simulink model "sm_car_"  (R2026b)
settings: Solver=ode23t  StopTime=100  MaxStep=0.4  AbsTol=1e-3  EnableMultiTasking=on
PreLoadFcn:
  | % Due to usability issue in Repeating Sequence block
  | warning('off','Simulink:Masking:Invalid');
  | 
  | % Eliminate unnecessary warnings in inactive variants
  | % Warnings generated only if you click through inactive variant
  | warning('off','MATLAB:nonExistentField');
  | warning('off','Simulink:Parameters:BlkParamUndefined');
PostLoadFcn:
  | set_param([bdroot '/Vehicle'],'popup_trailer','Off')
  | warning('off','sm:sli:setup:compile:LocalSolverNotSupported')
  | %sm_car_config_maneuver(bdroot,'WOT Braking');
  | sm_car_config_vehicle(bdroot,'false');
  | sm_car_config_logging(bdroot);
InitFcn:
  | sm_car_config_camera;
  | Vehicle = sm_car_vehcfg_checkConfig(Vehicle);
  | sm_car_check_tire_model(bdroot);
StartFcn:
  | tic;
StopFcn:
  | Elapsed_Sim_Time = toc;
  | % disp(['Elapsed Sim Time = ' num2str(Elapsed_Sim_Time)]);
undefined symbols (not defined in the file or in its folder): acc_theta, accel_ramp_rate, Axle1D, AxleIn, Camera, Control, Driver, Init, Maneuver, Pedal, Scene, ShaftL1, ShaftL2, ShaftR1, ShaftR2, Visual, X, xy_data_car_side, Y, Z
libraries: sm_lib x290, fl_lib x171, nesl_utility x144, simulink x60, simulink_extras x14, sdl_lib x14, SimscapeFluids_lib x7, Damper_Element x4, Tire_1x2x x4, ee_lib x3, Scene_Utilities x3, sharedTrackingLibrary x2
(part 4 of 22)

== system sm_car_/Controller/TrqVec_FLC_V3 ==
  DrvBus : Inport
  VehBus : Inport  Port=2
  Brake Control : Subsystem  Variant=on  VariantControlMode=label  VariantControl=Variant1  LabelModeActiveChoice=Pedal  mask{popup_brake_control=Pedal, abs_tire_radiusF=Vehicle.Chassis.Tire.tire_radius.Value, abs_tire_radiusR=Vehicle.Chassis.Tire.tire_radius.Value}
      mask prompts: popup_brake_control "Control Type"; abs_tire_radiusF "Tire Radius Front (m)"; abs_tire_radiusR "Tire Radius Rear (m)"
      mask init:
      | set_param(gcb,'LabelModeActiveChoice',get_param(gcb,'popup_brake_control'));
      settings: AttributesFormatString=%<ActiveVariant>
      mask TypeOptions popup_brake_control: Pedal | Pressure | ABS
      mask Display: disp(' ');
  Bus Creator1 : BusCreator  Inputs=4
  Bus Creator2 : BusCreator  Inputs=6
  Bus Selector : BusSelector  OutputSignals=Chassis.Body.CG.vx
  Bus Selector1 : BusSelector  OutputSignals=aSteerWheel,rAccelPedal,rBrakePedal
  Driveline Control : Subsystem
  Power Control : Subsystem  mask{Control=Control}
      mask prompts: Control "Control Parameters"
  Spring Damper : Subsystem
  Susp : Subsystem  mask{Steer=Control.Steer}
      mask prompts: Steer "Steer (structure)"
  CtrlBus : Outport  VectorParamsAs1DForOutWhenUnconnected=off
  wires:
  DrvBus/1 -> Bus Selector1/1
  Bus Creator2/1 -> CtrlBus/1  "CtrlBus"
  Bus Selector1/3 -> Brake Control/1("rBrakePedal ")  "<rBrakePedal>"
  Bus Selector1/2 -> Power Control/1(rAccelPedal)  "<rAccelPedal>"
  Spring Damper/2(Spring) -> Bus Creator1/4
  Power Control/1(Power) -> Bus Creator2/2  "Power"
  Driveline Control/1(Driveline) -> Bus Creator2/4
  Spring Damper/1(Damper) -> Bus Creator1/3
  Bus Creator1/1 -> Bus Creator2/1  "Chassis"
  Brake Control/1(" Brakes") -> Bus Creator2/5
  Susp/1(SuspA1) -> Bus Creator1/1
  VehBus/1 -> Power Control/2(VehBus), Brake Control/2("VehBus "), Bus Selector/1
  Susp/2(SuspA2) -> Bus Creator1/2
  Bus Selector1/1 -> Power Control/3(aSteerWheel), Susp/1(aSteerWheel)  "<aSteerWheel>"
  Bus Selector/1 -> Susp/2(vx)  "<vx>"
  Power Control/2(Meas) -> Bus Creator2/3  "Control"

== system sm_car_/Driver/Closed Loop ==
  VehBus : Inport
  Obs : Inport  Port=2
  Bus Selector : BusSelector  OutputSignals=Chassis.Body.CG.vx
  Bus Selector2 : BusSelector  OutputSignals=dist
  Driver : Subsystem  mask(Driver Behavior){Driver=Driver}
      mask help: Models driver behavior to follow prescribed vehicle trajectory, including path and speed.
  Driver Override : Subsystem  Variant=on  VariantControlMode=label  VariantControl=Choice  LabelModeActiveChoice=None  mask(Override Driver Commands){popup_driver_override=None}
      mask prompts: popup_driver_override "Driver Override"
      mask help: Override closed-loop driver commands with open-loop inputs. Can be applied to steering wheel, accelerator pedal. or brake pedal.
      mask init:
      | curblk = gcb;
      | 
      | set_param(curblk,'LabelModeActiveChoice',get_param(curblk,'popup_driver_override'));
      mask TypeOptions popup_driver_override: None | Override
  Maneuver : Subsystem  mask(Maneuver Follow Trajectory){Maneuver=Maneuver, Value=Maneuver.vGain.Value, popup_window=Yes}
      mask prompts: Value "vGain"; popup_window "Check only window of trajectory"
      mask help: Determines target pose to follow prescribed trajectory. Prescribed trajectory is vehicle pose (x, y, theta) and speed along the path to be followed. Optional visual of target pose is also provided.
      mask init:
      | if(strcmpi(get_param(gcb,'popup_window'),'yes'))
      |     set_param([gcb '/window only'],'Value','1');
      | else
      |     set_param([gcb '/window only'],'Value','0');
      | end
      mask TypeOptions Value: Target Speed Gain/Value
      mask TypeOptions popup_window: No | Yes
  Override : Subsystem  Variant=on  VariantControlMode=label  VariantControl=Variant1  LabelModeActiveChoice=None  mask(Driver Override){popup_override_type=None}
      mask prompts: popup_override_type "Override Type"
      mask help: Optionally override driver commands based on objects in scene. For example, the state of a traffic light can override driver commands to follow a prescribed speed trajectory.
      mask init:
      | set_param(gcb,'LabelModeActiveChoice',strrep(get_param(gcb,'popup_override_type'),' ','_'));
      settings: AttributesFormatString=%<LabelModeActiveChoice>
      mask TypeOptions popup_override_type: None | Track Mallory Park Obstacle
      mask Display: disp(' ');
  Scopes : Subsystem
  Terminator : Terminator
  Transfer Fcn : TransferFcn  Denominator=[0.1 1]
  DrvBus : Outport  VectorParamsAs1DForOutWhenUnconnected=off
  wires:
  Obs/1 -> Override/2("Obs ")
  Bus Selector2/1 -> Transfer Fcn/1  "<dist>"
  Transfer Fcn/1 -> Override/1("dist ")
  Driver/1(DrvBus) -> Driver Override/1(In), Scopes/4(DrvBus)
  Driver Override/1(DrvBus) -> DrvBus/1
  Maneuver/3(simres) -> Terminator/1
  Maneuver/1(Ref) -> Bus Selector2/1, Scopes/2(Ref), Driver/2(Ref)
  Maneuver/2(CurPose) -> Scopes/3(CurPose), Driver/3(CurPose)
  VehBus/1 -> Bus Selector/1, Maneuver/1(VehBus)
  Bus Selector/1 -> Scopes/1(<vx>), Driver/1(vx)  "<vx>"
  Override/1(" Ovr") -> Maneuver/2(Override)

== system sm_car_/Driver/Closed Loop1 ==
  VehBus : Inport
  Obs : Inport  Port=2
  Bus Selector2 : BusSelector  OutputSignals=dist
  Driver : Subsystem  mask(Driver Behavior){Driver=Driver}
      mask help: Models driver behavior to follow prescribed vehicle trajectory, including path and speed.
  Driver Override : Subsystem  Variant=on  VariantControlMode=label  VariantControl=Choice  LabelModeActiveChoice=None  mask(Override Driver Commands){popup_driver_override=None}
      mask prompts: popup_driver_override "Driver Override"
      mask help: Override closed-loop driver commands with open-loop inputs. Can be applied to steering wheel, accelerator pedal. or brake pedal.
      mask init:
      | curblk = gcb;
      | 
      | set_param(curblk,'LabelModeActiveChoice',get_param(curblk,'popup_driver_override'));
      mask TypeOptions popup_driver_override: None | Override
  Maneuver : Subsystem  mask(Maneuver Follow Trajectory){Maneuver=Maneuver, popup_window=Yes}
      mask prompts: popup_window "Check only window of trajectory"
      mask help: Determines target pose to follow prescribed trajectory. Prescribed trajectory is vehicle pose (x, y, theta) and speed along the path to be followed. Optional visual of target pose is also provided.
      mask init:
      | if(strcmpi(get_param(gcb,'popup_window'),'yes'))
      |     set_param([gcb '/window only'],'Value','1');
      | else
      |     set_param([gcb '/window only'],'Value','0');
      | end
      mask TypeOptions popup_window: No | Yes
  Override : Subsystem  Variant=on  VariantControlMode=label  VariantControl=Variant1  LabelModeActiveChoice=None  mask(Driver Override){popup_override_type=None}
      mask prompts: popup_override_type "Override Type"
      mask help: Optionally override driver commands based on objects in scene. For example, the state of a traffic light can override driver commands to follow a prescribed speed trajectory.
      mask init:
      | set_param(gcb,'LabelModeActiveChoice',strrep(get_param(gcb,'popup_override_type'),' ','_'));
      settings: AttributesFormatString=%<LabelModeActiveChoice>
      mask TypeOptions popup_override_type: None | Track Mallory Park Obstacle
      mask Display: disp(' ');
  Scopes : Subsystem
  Terminator : Terminator
  Terminator1 : Terminator
  Transfer Fcn : TransferFcn  Denominator=[0.1 1]
  DrvBus : Outport  VectorParamsAs1DForOutWhenUnconnected=off
  wires:
  Override/1(" Ovr") -> Maneuver/2(Override)
  VehBus/1 -> Maneuver/1(VehBus)
  Maneuver/3(CurPose) -> Driver/3(CurPose), Scopes/3(CurPose)
  Maneuver/2(Ref) -> Driver/2(Ref), Scopes/2(Ref), Bus Selector2/1
  Maneuver/4(Preview) -> Terminator/1
  Driver Override/1(DrvBus) -> DrvBus/1
  Driver/1(DrvBus) -> Scopes/4(DrvBus), Driver Override/1(In)
  Transfer Fcn/1 -> Override/1("dist ")
  Bus Selector2/1 -> Transfer Fcn/1  "<dist>"
  Obs/1 -> Override/2("Obs ")
  Maneuver/1(vx) -> Scopes/1(<vx>), Driver/1(vx)
  Maneuver/5(simres) -> Terminator1/1

== system sm_car_/Driver/Open Loop ==
  VehBus : Inport
  Obs : Inport  Port=2
  Open Loop : Subsystem  mask{Maneuver=Maneuver}
      mask init:
      | X = [0 0];
      | Y = [0 0];
  Terminator : Terminator
  Terminator1 : Terminator
  DrvBus : Outport  VectorParamsAs1DForOutWhenUnconnected=off
  wires:
  Obs/1 -> Terminator1/1
  VehBus/1 -> Terminator/1
  Open Loop/1(DrvBus) -> DrvBus/1

== system sm_car_/Road/Ground ==
  gz : Inport
  uvec : Inport  Port=2
  TyreScaling FL : Inport  Port=3
  TyreScaling FR : Inport  Port=4
  TyreScaling RL : Inport  Port=5
  TyreScaling RR : Inport  Port=6
  Bus Creator{,1..3} (4 alike) : BusCreator  Inputs=3
  Bus Selector : BusSelector  OutputSignals=L1,R1,L2,R2
  Bus Selector1 : BusSelector  OutputSignals=L1,R1,L2,R2
  Gain{,1..7} (8 alike) : Gain
  Signal Specification1 : SignalSpecification  Unit=m
  L1 : Outport  VectorParamsAs1DForOutWhenUnconnected=off
  R1 : Outport  Port=2  VectorParamsAs1DForOutWhenUnconnected=off
  L2 : Outport  Port=3  VectorParamsAs1DForOutWhenUnconnected=off
  R2 : Outport  Port=4  VectorParamsAs1DForOutWhenUnconnected=off
  wires:
  Bus Creator/1 -> L1/1  "L1"
  Bus Creator1/1 -> R1/1  "R1"
  Gain1/1 -> Bus Creator1/1  "gz"
  TyreScaling FL/1 -> Bus Creator/3  "TyreScaling"
  Bus Creator3/1 -> R2/1  "R2"
  gz/1 -> Signal Specification1/1
  Gain3/1 -> Bus Creator3/1  "gz"
  Bus Creator2/1 -> L2/1  "L2"
  Signal Specification1/1 -> Bus Selector/1
  Gain2/1 -> Bus Creator2/1  "gz"
  TyreScaling FR/1 -> Bus Creator1/3  "TyreScaling"
  TyreScaling RL/1 -> Bus Creator2/3  "TyreScaling"
  TyreScaling RR/1 -> Bus Creator3/3  "TyreScaling"
  Bus Selector/1 -> Gain/1  "<L1>"
  Gain/1 -> Bus Creator/1  "gz"
  Bus Selector/2 -> Gain1/1  "<R1>"
  Bus Selector/3 -> Gain2/1  "<L2>"
  Bus Selector/4 -> Gain3/1  "<R2>"
  uvec/1 -> Bus Selector1/1
  Bus Selector1/1 -> Gain4/1  "<L1>"
  Bus Selector1/2 -> Gain5/1  "<R1>"
  Bus Selector1/3 -> Gain6/1  "<L2>"
  Bus Selector1/4 -> Gain7/1  "<R2>"
  Gain4/1 -> Bus Creator/2  "uvec"
  Gain5/1 -> Bus Creator1/2  "uvec"
  Gain6/1 -> Bus Creator2/2  "uvec"
  Gain7/1 -> Bus Creator3/2  "uvec"

== system sm_car_/Road/Input fWindCar ==
  Bus Creator1 : BusCreator  Inputs=3
  Demux : Demux  Outputs=3
  Step : Step  Time=dWind  FinalValue=fWind  SampleTime=0
  Step1 : Step  Time=dWind+tWind  FinalValue=fWind  SampleTime=0
  Sum : Sum  Inputs=|+-
  fWind : Outport  VectorParamsAs1DForOutWhenUnconnected=off
  wires:
  Demux/2 -> Bus Creator1/2  "fy"
  Demux/1 -> Bus Creator1/1  "fx"
  Demux/3 -> Bus Creator1/3  "fz"
  Bus Creator1/1 -> fWind/1
  Step/1 -> Sum/1
  Step1/1 -> Sum/2
  Sum/1 -> Demux/1

== system sm_car_/Road/Input fWindTrailer ==
  Bus Creator1 : BusCreator  Inputs=3
  Demux : Demux  Outputs=3
  Scope : Scope
      settings: ActiveDisplayYMinimum=-1  ActiveDisplayYMaximum=1
  Step : Step  Time=dWind  FinalValue=fWind  SampleTime=0
  Step1 : Step  Time=dWind+tWind  FinalValue=fWind  SampleTime=0
  Sum : Sum  Inputs=|+-
  fWind : Outport  VectorParamsAs1DForOutWhenUnconnected=off
  wires:
  Bus Creator1/1 -> fWind/1
  Demux/3 -> Bus Creator1/3  "fz"
  Demux/1 -> Bus Creator1/1  "fx"
  Demux/2 -> Bus Creator1/2  "fy"
  Sum/1 -> Scope/1, Demux/1  "fxyz"
  Step1/1 -> Sum/2
  Step/1 -> Sum/1

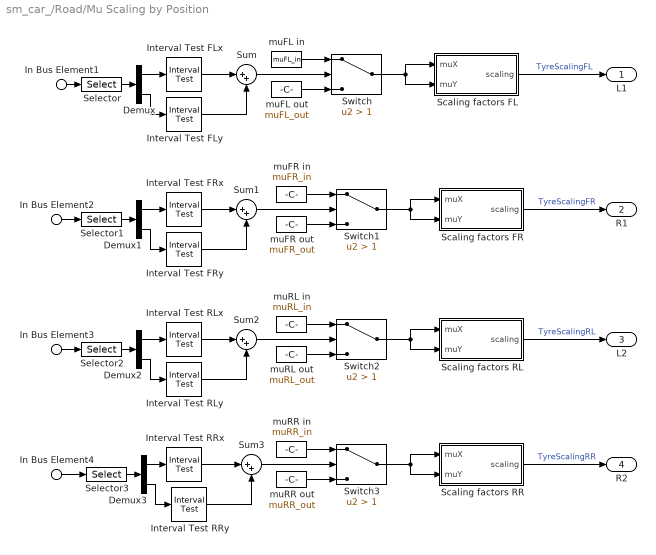
== system sm_car_/Road/Mu Scaling by Position ==
  In Bus Element1 : Inport  PortName=Chassis  Element=WhlL1.xyz
  In Bus Element2 : Inport  PortName=Chassis  Element=WhlR1.xyz
  In Bus Element3 : Inport  PortName=Chassis  Element=WhlL2.xyz
  In Bus Element4 : Inport  PortName=Chassis  Element=WhlR2.xyz
  Demux{,1..3} (4 alike) : Demux  Outputs=2
  Interval Test FLx : simulink/Logic and Bit Operations/Interval Test  IntervalClosedRight=on  uplimit=intvX_FL_end  IntervalClosedLeft=on  lowlimit=intvX_FL_start  OutDataTypeStr=uint8
  Interval Test FLy : simulink/Logic and Bit Operations/Interval Test  IntervalClosedRight=on  uplimit=intvY_FL_end  IntervalClosedLeft=on  lowlimit=intvY_FL_start  OutDataTypeStr=uint8
  Interval Test FRx : simulink/Logic and Bit Operations/Interval Test  IntervalClosedRight=on  uplimit=intvX_FR_end  IntervalClosedLeft=on  lowlimit=intvX_FR_start  OutDataTypeStr=uint8
  Interval Test FRy : simulink/Logic and Bit Operations/Interval Test  IntervalClosedRight=on  uplimit=intvY_FR_end  IntervalClosedLeft=on  lowlimit=intvY_FR_start  OutDataTypeStr=uint8
  Interval Test RLx : simulink/Logic and Bit Operations/Interval Test  IntervalClosedRight=on  uplimit=intvX_RL_end  IntervalClosedLeft=on  lowlimit=intvX_RL_start  OutDataTypeStr=uint8
  Interval Test RLy : simulink/Logic and Bit Operations/Interval Test  IntervalClosedRight=on  uplimit=intvY_RL_end  IntervalClosedLeft=on  lowlimit=intvY_RL_start  OutDataTypeStr=uint8
  Interval Test RRx : simulink/Logic and Bit Operations/Interval Test  IntervalClosedRight=on  uplimit=intvX_RR_end  IntervalClosedLeft=on  lowlimit=intvX_RR_start  OutDataTypeStr=uint8
  Interval Test RRy : simulink/Logic and Bit Operations/Interval Test  IntervalClosedRight=on  uplimit=intvY_RR_end  IntervalClosedLeft=on  lowlimit=intvY_RR_start  OutDataTypeStr=uint8
  Scaling factors FL : Subsystem  mask{LKX=1, LKY=1, LKYC=1, LTR=1, LKZC=1}
      mask prompts: LKX "longitudinal slip stiffness"; LKY "cornering stiffness"; LKYC "camber stiffness"; LTR "pneumatic trail"; LKZC "camber torque stiffness"
  Scaling factors FR : Subsystem  mask{LKX=1, LKY=1, LKYC=1, LTR=1, LKZC=1}
      mask prompts: LKX "longitudinal slip stiffness"; LKY "cornering stiffness"; LKYC "camber stiffness"; LTR "pneumatic trail"; LKZC "camber torque stiffness"
  Scaling factors RL : Subsystem  mask{LKX=1, LKY=1, LKYC=1, LTR=1, LKZC=1}
      mask prompts: LKX "longitudinal slip stiffness"; LKY "cornering stiffness"; LKYC "camber stiffness"; LTR "pneumatic trail"; LKZC "camber torque stiffness"
  Scaling factors RR : Subsystem  mask{LKX=1, LKY=1, LKYC=1, LTR=1, LKZC=1}
      mask prompts: LKX "longitudinal slip stiffness"; LKY "cornering stiffness"; LKYC "camber stiffness"; LTR "pneumatic trail"; LKZC "camber torque stiffness"
  Selector{,1..3} (4 alike) : Selector  InputPortWidth=3  IndexOptions=Index vector (dialog)  Indices=[1 2]  OutputSizes=1  RuntimeRangeChecks=off
  Sum{,1..3} (4 alike) : Sum  Inputs=|++
  Switch : Switch  Criteria=u2 > Threshold  Threshold=1  ZeroCross=off  SaturateOnIntegerOverflow=off  InputSameDT=off
  Switch1 : Switch  Criteria=u2 > Threshold  Threshold=1  SaturateOnIntegerOverflow=off  InputSameDT=off
  Switch2 : Switch  Criteria=u2 > Threshold  Threshold=1  SaturateOnIntegerOverflow=off  InputSameDT=off
  Switch3 : Switch  Criteria=u2 > Threshold  Threshold=1  SaturateOnIntegerOverflow=off  InputSameDT=off
  muFL in : Constant  Value=muFL_in
  muFL out : Constant  Value=muFL_out
  muFR in : Constant  Value=muFR_in
  muFR out : Constant  Value=muFR_out
  muRL in : Constant  Value=muRL_in
  muRL out : Constant  Value=muRL_out
  muRR in : Constant  Value=muRR_in
  muRR out : Constant  Value=muRR_out
  L1 : Outport  VectorParamsAs1DForOutWhenUnconnected=off
  R1 : Outport  Port=2  VectorParamsAs1DForOutWhenUnconnected=off
  L2 : Outport  Port=3  VectorParamsAs1DForOutWhenUnconnected=off
  R2 : Outport  Port=4  VectorParamsAs1DForOutWhenUnconnected=off
  wires:
  Demux/1 -> Interval Test FLx/1
  Interval Test RRx/1 -> Sum3/1
  Demux3/2 -> Interval Test RRy/1
  Demux3/1 -> Interval Test RRx/1
  Sum3/1 -> Switch3/2
  Selector3/1 -> Demux3/1
  In Bus Element4/1 -> Selector3/1
  Interval Test RRy/1 -> Sum3/2
  Demux2/2 -> Interval Test RLy/1
  Selector2/1 -> Demux2/1
  Demux2/1 -> Interval Test RLx/1
  Interval Test RLy/1 -> Sum2/2
  Sum2/1 -> Switch2/2
  In Bus Element3/1 -> Selector2/1
  Interval Test RLx/1 -> Sum2/1
  Interval Test FRy/1 -> Sum1/2
  Selector1/1 -> Demux1/1
  Demux1/2 -> Interval Test FRy/1
  Sum1/1 -> Switch1/2
  Demux1/1 -> Interval Test FRx/1
  Interval Test FRx/1 -> Sum1/1
  Interval Test FLx/1 -> Sum/1
  Interval Test FLy/1 -> Sum/2
  Sum/1 -> Switch/2
  Demux/2 -> Interval Test FLy/1
  Selector/1 -> Demux/1
  muRR out/1 -> Switch3/3
  muRR in/1 -> Switch3/1
  Switch3/1 -> Scaling factors RR/2(muY), Scaling factors RR/1(muX)
  Scaling factors RR/1(scaling) -> R2/1  "TyreScalingRR"
  Scaling factors RL/1(scaling) -> L2/1  "TyreScalingRL"
  Switch2/1 -> Scaling factors RL/1(muX), Scaling factors RL/2(muY)
  muRL in/1 -> Switch2/1
  muRL out/1 -> Switch2/3
  muFR out/1 -> Switch1/3
  In Bus Element2/1 -> Selector1/1
  muFR in/1 -> Switch1/1
  Switch1/1 -> Scaling factors FR/2(muY), Scaling factors FR/1(muX)
  Scaling factors FR/1(scaling) -> R1/1  "TyreScalingFR"
  Scaling factors FL/1(scaling) -> L1/1  "TyreScalingFL"
  Switch/1 -> Scaling factors FL/1(muX), Scaling factors FL/2(muY)
  muFL out/1 -> Switch/3
  muFL in/1 -> Switch/1
  In Bus Element1/1 -> Selector/1

== system sm_car_/Road/Road Surface Height ==
  Chassis : Inport
  None : Subsystem  VariantControl=None
  gz : Outport  VectorParamsAs1DForOutWhenUnconnected=off
  uvec : Outport  Port=2  VectorParamsAs1DForOutWhenUnconnected=off

== system sm_car_/Scopes/Combined Tire Usage ==
  VehBus : Inport
  Bus Creator : BusCreator  Inputs=4
  Bus Selector10 : BusSelector  OutputSignals=Chassis.WhlL1.Fx,Chassis.WhlL1.Fy,Chassis.WhlL1.Fz,Chassis.WhlL1.rMuX,Chassis.WhlL1.rMuY
  Bus Selector11 : BusSelector  OutputSignals=Chassis.WhlR1.Fx,Chassis.WhlR1.Fy,Chassis.WhlR1.Fz,Chassis.WhlR1.rMuX,Chassis.WhlR1.rMuY
  Bus Selector12 : BusSelector  OutputSignals=Chassis.WhlL2.Fx,Chassis.WhlL2.Fy,Chassis.WhlL2.Fz,Chassis.WhlL2.rMuX,Chassis.WhlL2.rMuY
  Bus Selector13 : BusSelector  OutputSignals=Chassis.WhlR2.Fx,Chassis.WhlR2.Fy,Chassis.WhlR2.Fz,Chassis.WhlR2.rMuX,Chassis.WhlR2.rMuY
  FL_Fcomb : Subsystem
  FR_Fcomb : Subsystem
  RL_Fcomb : Subsystem
  RR_Fcomb : Subsystem
  Fcomb% : Outport
  wires:
  FL_Fcomb/1(Fcomb%) -> Bus Creator/1  "FL_Fcomb%"
  Bus Selector11/4 -> FR_Fcomb/4(<rMuX>)  "<rMuX>"
  Bus Selector13/5 -> RR_Fcomb/5(<rMuY>)  "<rMuY>"
  Bus Selector12/1 -> RL_Fcomb/1(<Fx>)  "<Fx>"
  Bus Selector11/2 -> FR_Fcomb/2(<Fy>)  "<Fy>"
  Bus Selector10/4 -> FL_Fcomb/4(<rMuX>)  "<rMuX>"
  Bus Selector10/3 -> FL_Fcomb/3(<Fz>)  "<Fz>"
  Bus Selector12/2 -> RL_Fcomb/2(<Fy>)  "<Fy>"
  Bus Selector13/3 -> RR_Fcomb/3(<Fz>)  "<Fz>"
  Bus Selector12/4 -> RL_Fcomb/4(<rMuX>)  "<rMuX>"
  Bus Selector11/3 -> FR_Fcomb/3(<Fz>)  "<Fz>"
  VehBus/1 -> Bus Selector13/1, Bus Selector12/1, Bus Selector11/1, Bus Selector10/1
  Bus Selector13/1 -> RR_Fcomb/1(<Fx>)  "<Fx>"
  Bus Selector13/4 -> RR_Fcomb/4(<rMuX>)  "<rMuX>"
  Bus Selector11/1 -> FR_Fcomb/1(<Fx>)  "<Fx>"
  RR_Fcomb/1(Fcomb%) -> Bus Creator/4  "RR_Fcomb%"
  FR_Fcomb/1(Fcomb%) -> Bus Creator/2  "FR_Fcomb%"
  Bus Selector10/2 -> FL_Fcomb/2(<Fy>)  "<Fy>"
  Bus Selector12/3 -> RL_Fcomb/3(<Fz>)  "<Fz>"
  Bus Selector10/1 -> FL_Fcomb/1(<Fx>)  "<Fx>"
  RL_Fcomb/1(Fcomb%) -> Bus Creator/3  "RL_Fcomb%"
  Bus Selector11/5 -> FR_Fcomb/5(<rMuY>)  "<rMuY>"
  Bus Selector10/5 -> FL_Fcomb/5(<rMuY>)  "<rMuY>"
  Bus Selector12/5 -> RL_Fcomb/5(<rMuY>)  "<rMuY>"
  Bus Selector13/2 -> RR_Fcomb/2(<Fy>)  "<Fy>"
  Bus Creator/1 -> Fcomb%/1

== system sm_car_/Scopes/Lateral Tire Usage ==
  VehBus : Inport
  Bus Creator : BusCreator  Inputs=4
  Bus Selector9 : BusSelector  OutputSignals=Chassis.WhlL1.Fy,Chassis.WhlL1.rMuY,Chassis.WhlL1.Fz,Chassis.WhlR1.Fy,Chassis.WhlR1.rMuY,Chassis.WhlR1.Fz,Chassis.WhlL2.Fy,Chassis.WhlL2.rMuY,Chassis.WhlL2.Fz,Chassis.WhlR2.Fy,Chassis.WhlR2.rMuY,Chassis.WhlR2.Fz
  FL_Y : Subsystem
  FR_Y : Subsystem
  RL_Y : Subsystem
  RR_Y : Subsystem
  Fy% : Outport
  wires:
  Bus Selector9/9 -> RL_Y/3(<Fz>)  "<Fz>"
  Bus Selector9/11 -> RR_Y/2(<rMuY>)  "<rMuY>"
  RR_Y/1(Fy%) -> Bus Creator/4  "RR_FY%"
  Bus Selector9/8 -> RL_Y/2(<rMuY>)  "<rMuY>"
  VehBus/1 -> Bus Selector9/1
  Bus Selector9/5 -> FR_Y/2(<rMuY>)  "<rMuY>"
  Bus Selector9/3 -> FL_Y/3(<Fz>)  "<Fz>"
  RL_Y/1(Fy%) -> Bus Creator/3  "RL_FY%"
  Bus Selector9/6 -> FR_Y/3(<Fz>)  "<Fz>"
  Bus Selector9/12 -> RR_Y/3(<Fz>)  "<Fz>"
  FR_Y/1(Fy%) -> Bus Creator/2  "FR_FY%"
  Bus Selector9/1 -> FL_Y/1(<Fy>)  "<Fy>"
  FL_Y/1(Fy%) -> Bus Creator/1  "FL_FY%"
  Bus Selector9/7 -> RL_Y/1(<Fy>)  "<Fy>"
  Bus Selector9/2 -> FL_Y/2(<rMuY>)  "<rMuY>"
  Bus Selector9/4 -> FR_Y/1(<Fy>)  "<Fy>"
  Bus Selector9/10 -> RR_Y/1(<Fy>)  "<Fy>"
  Bus Creator/1 -> Fy%/1

== system sm_car_/Scopes/Longitudinal Tire Usage ==
  VehBus : Inport
  Bus Creator : BusCreator  Inputs=2
  Bus Selector8 : BusSelector  OutputSignals=Chassis.WhlL2.Fx,Chassis.WhlL2.rMuX,Chassis.WhlL2.Fz,Chassis.WhlR2.Fx,Chassis.WhlR2.rMuX,Chassis.WhlR2.Fz
  RL_X : Subsystem
  RR_X : Subsystem
  Fx% : Outport
  wires:
  Bus Selector8/1 -> RL_X/1(<Fx>)  "<Fx>"
  Bus Selector8/5 -> RR_X/2(<rMuX>)  "<rMuX>"
  RL_X/1(Fx%) -> Bus Creator/1  "RL_FX%"
  Bus Selector8/6 -> RR_X/3(<Fz>)  "<Fz>"
  Bus Selector8/4 -> RR_X/1(<Fx>)  "<Fx>"
  Bus Selector8/2 -> RL_X/2(<rMuX>)  "<rMuX>"
  RR_X/1(Fx%) -> Bus Creator/2  "RR_FX%"
  VehBus/1 -> Bus Selector8/1
  Bus Selector8/3 -> RL_X/3(<Fz>)  "<Fz>"
  Bus Creator/1 -> Fx%/1

== system sm_car_/Scopes/Stability Factor ==
  VehBus : Inport
  Abs4 : Abs  SaturateOnIntegerOverflow=off
  Bus Selector2 : BusSelector  OutputSignals=Chassis.Body.CG.gy
  Compare To Constant1 : simulink/Logic and Bit Operations/Compare To Constant  relop=>=  const=0.4  OutDataTypeStr=boolean
  Understeer Gradient Calculation : Subsystem
  K : Outport
  wires:
  VehBus/1 -> Understeer Gradient Calculation/1(VehBus), Bus Selector2/1
  Understeer Gradient Calculation/1(K) -> K/1  "K"
  Bus Selector2/1 -> Abs4/1  "<gy>"
  Compare To Constant1/1 -> Understeer Gradient Calculation/Enable
  Abs4/1 -> Compare To Constant1/1

== system sm_car_/Scopes/Subsystem ==
  In1 : Inport
  Bus Selector4 : BusSelector  OutputSignals=Chassis.Body.CG.vx,Chassis.Body.CG.vy,World.vx,World.vy,World.x,World.y
  Mux : Mux  Inputs=2
  Mux1 : Mux  Inputs=2
  Mux2 : Mux  Inputs=2
  Vel in xy plane : Fcn  Expr=sqrt(u(1)^2+u(2)^2)
  Vel in xy plane1 : Fcn  Expr=sqrt(u(1)^2+u(2)^2)
  Vel in xy plane2 : Fcn  Expr=sqrt(u(1)^2+u(2)^2)
  vBody : Outport  VectorParamsAs1DForOutWhenUnconnected=off
  vWorld : Outport  Port=2  VectorParamsAs1DForOutWhenUnconnected=off
  xWorld : Outport  Port=3  VectorParamsAs1DForOutWhenUnconnected=off
  wires:
  Bus Selector4/3 -> Mux1/1  "<vx>"
  Bus Selector4/4 -> Mux1/2  "<vy>"
  Bus Selector4/1 -> Mux/1  "<vx>"
  Vel in xy plane1/1 -> vWorld/1  "speed"
  In1/1 -> Bus Selector4/1
  Mux1/1 -> Vel in xy plane1/1
  Mux/1 -> Vel in xy plane/1
  Vel in xy plane/1 -> vBody/1  "speed"
  Bus Selector4/2 -> Mux/2  "<vy>"
  Mux2/1 -> Vel in xy plane2/1
  Bus Selector4/6 -> Mux2/2  "<y>"
  Bus Selector4/5 -> Mux2/1  "<x>"
  Vel in xy plane2/1 -> xWorld/1  "speed"

== system sm_car_/Scopes/Yaw Reference ==
  aSteerWheel : Inport
  a_y : Inport  Port=2
  v_x : Inport  Port=3
  Compare To Constant : simulink/Logic and Bit Operations/Compare To Constant  relop=>  const=0  OutDataTypeStr=boolean
  Subsystem : Subsystem
  nYaw_Ref : Outport
  wires:
  aSteerWheel/1 -> Subsystem/2(aSteerWheel)  "aSteerWheel [rad]"
  v_x/1 -> Subsystem/1(v_x), Compare To Constant/1
  a_y/1 -> Subsystem/3(a_y)
  Subsystem/1(y) -> nYaw_Ref/1
  Compare To Constant/1 -> Subsystem/Enable

== system sm_car_/Vehicle/Trailer ==
  "RdBus " : Inport
  "DrvBus " : Inport  Port=2
  "CtrlBus " : Inport  Port=3
  None : Subsystem  VariantControl=None
  " C" : PMIOPort  Side=Left
  " W" : PMIOPort  Port=2  Side=Left
  " Hitch" : PMIOPort  Port=3  Side=Right
  " VehBus" : Outport  VectorParamsAs1DForOutWhenUnconnected=off

== system sm_car_/Vehicle/Vehicle ==
  In Bus Element2 : Inport  PortName=RdBus
  In Bus Element : Inport  Port=2  PortName=DrvBus
  In Bus Element3 : Inport  Port=2  PortName=DrvBus
  In Bus Element6 : Inport  Port=3  PortName=CtrlBus  Element=Brakes
  In Bus Element5 : Inport  Port=3  PortName=CtrlBus  Element=Chassis
  In Bus Element1 : Inport  Port=3  PortName=CtrlBus  Element=Power
  In Bus Element4 : Inport  Port=3  PortName=CtrlBus  Element=Driveline
  A1 to World : Subsystem  mask(Body to World){Init=Init.Chassis, SpecifyPosTarget=off}
      mask prompts: Init "Initial Values"; SpecifyPosTarget "Specify Position Target"
      mask help: Models the connection between the vehicle body and world. Permits 6 degrees of freedom and sets the initial position, orientation, and speed of the vehicle body.
      mask init:
      | initial_aveh = [Init.aChassis.Value(3) Init.aChassis.Value(2) Init.aChassis.Value(1)];
      | rotmat_ypr = sm_car_yawpitchroll_to_rotmat(Init.aChassis.Value(3),Init.aChassis.Value(2),Init.aChassis.Value(1));
      | initial_vveh = rotmat_ypr*(Init.vChassis.Value)';
      | 
      | sptState = get_param(gcb,'SpecifyPosTarget');
      | 
      | set_param([gcb '/Body World Joint'],...
      |         'PxPositionTargetSpecify',sptState,...
      |         'PyPositionTargetSpecify',sptState,...
      |         'PzPositionTargetSpecify',sptState,...
      |         'SphPositionTargetSpecify',sptState,...
      |         'PxVelocityTargetSpecify',sptState,...
      |         'PyVelocityTargetSpecify',sptState,...
      |         'PzVelocityTargetSpecify',sptState...
      |         );
      mask Help: web('sm_car_doc_body_to_world.html')
  A2 to World : Subsystem  mask(Body to World){Init=Init.Chassis, SpecifyPosTarget=off}
      mask prompts: Init "Initial Values"; SpecifyPosTarget "Specify Position Target"
      mask help: Models the connection between the vehicle body and world. Permits 6 degrees of freedom and sets the initial position, orientation, and speed of the vehicle body.
      mask init: same as sm_car_/Vehicle/Vehicle/A1 to World
      mask Help: web('sm_car_doc_body_to_world.html')
  Body to World : Subsystem  mask(Body to World){Init=Init.Chassis, SpecifyPosTarget=on}
      mask prompts: Init "Initial Values"; SpecifyPosTarget "Specify Position Target"
      mask help: Models the connection between the vehicle body and world. Permits 6 degrees of freedom and sets the initial position, orientation, and speed of the vehicle body.
      mask init: same as sm_car_/Vehicle/Vehicle/A1 to World
      mask Help: web('sm_car_doc_body_to_world.html')
  Brakes : Subsystem  Tag=PublishSubsystem  Variant=on  VariantControlMode=label  VariantControl=Variant1  LabelModeActiveChoice=PedalAbstract_DiscDisc  mask(Brake System){Brakes=Vehicle.Brakes, VariantLabel=Vehicle.Brakes.class.Value}
      mask prompts: Brakes "Brake Parameters"; VariantLabel "Variant Label"
      mask help: Select option and provide parameters for brakes. Option is chosen by string provided in Variant Label. The parameters for the selected option are contained in Brakes data structure.
      mask init:
      | curblk = gcb;
      | 
      | % Set variant for this block 
      | set_param(curblk,'LabelModeActiveChoice',VariantLabel);
      settings: AttributesFormatString=%<ActiveVariant>
  Chassis : Subsystem  Tag=PublishSubsystem  VariantControl=Chassis  mask(Chassis){Chassis=Vehicle.Chassis, Init=Init, mask_image_name=sm_car_vehicle_chassis_hamba_IMAGE.png, veh_index=veh_index}
      mask prompts: Chassis "Vehicle Parameters"; Init "Initial Values"; mask_image_name "Mask Image (string)"; veh_index "Vehicle Index (for tires)"
      mask help: Models vehicle chassis, with suspension, body, tires, springs, and dampers.
      mask Help: web('sm_car_doc_chassis.html')
      mask Display:
      | % Get image from BodyGeometry.class
      | % (active choice for Body Geometry subsystem)
      | temp_veh_bg_class = lower(get_param([gcb '/Body/Body Geometry'],'LabelModeActiveChoice'));
      | 
      | imagestr = (['sm_car_chassis_' temp_veh_bg_class '.png']);
      | if(~exist(imagestr))
      |     imagestr = ['sm_car_chassis_default.png'];
      | end
      | 
      | image(imagestr);
  Powertrain : Subsystem  mask(Powertrain, 2-Axle){Powertrain=Vehicle.Powertrain}
      mask prompts: Powertrain "Powertrain Parameters"
      mask help: Models power source and driveline for two-axle vehicles. The parameters for the selected options are contained in Powertrain data structure.
      mask Display: image('sm_car_vehicle_powertrain_IMAGE.png')
  C : PMIOPort  Side=Left
  W : PMIOPort  Port=2  Side=Left
  HitchR : PMIOPort  Port=3  Side=Left
  HitchF : PMIOPort  Port=4  Side=Right
  Out Bus Elemet5 : Outport  VectorParamsAs1DForOutWhenUnconnected=off  PortName=VehBus  Element=Chassis
  Out Bus Element : Outport  VectorParamsAs1DForOutWhenUnconnected=off  PortName=VehBus  Element=Brakes
  Out Bus Element1 : Outport  VectorParamsAs1DForOutWhenUnconnected=off  PortName=VehBus  Element=Driveline
  Out Bus Element2 : Outport  VectorParamsAs1DForOutWhenUnconnected=off  PortName=VehBus  Element=World
  Out Bus Element3 : Outport  VectorParamsAs1DForOutWhenUnconnected=off  PortName=VehBus  Element=Power
  Out Bus Element4 : Outport  VectorParamsAs1DForOutWhenUnconnected=off  PortName=VehBus  Element=Ride.A2
  Out Bus Element5 : Outport  VectorParamsAs1DForOutWhenUnconnected=off  PortName=VehBus  Element=Ride.A1
  wires:
  In Bus Element5/1 -> Chassis/3(CtrlBus)
  Brakes/1(" OutB") -> Out Bus Element/1
  Chassis/1(VehBus) -> [VehB], Out Bus Elemet5/1
  In Bus Element2/1 -> Chassis/2(RdBus)
  In Bus Element/1 -> Chassis/1(DrvBus)
  In Bus Element6/1 -> Brakes/2("CtrlBus ")
  Body to World/1(World) -> Out Bus Element2/1
  In Bus Element3/1 -> Brakes/1("DrvBus ")
  In Bus Element4/1 -> Powertrain/1(CtrlD)
  In Bus Element1/1 -> Powertrain/2(CtrlP)
  Powertrain/1(OutD) -> Out Bus Element1/1
  Powertrain/2(OutP) -> Out Bus Element3/1
  [VehB] -> Powertrain/3(VehB)
  A2 to World/1(World) -> Out Bus Element4/1
  A1 to World/1(World) -> Out Bus Element5/1
  connections:
  HitchR/RConn1 -- Chassis/LConn1
  C/RConn1 -- Body to World/LConn1 -- Chassis/RConn1
  Body to World/RConn1 -- A2 to World/RConn1 -- A1 to World/RConn1 -- W/RConn1
  Powertrain/LConn3 -- Chassis/LConn4 -- Brakes/LConn2
  Powertrain/RConn4 -- Chassis/RConn6 -- Brakes/RConn2
  Brakes/RConn1 -- Chassis/RConn5 -- Powertrain/RConn3
  Powertrain/LConn2 -- Chassis/LConn3 -- Brakes/LConn1
  HitchF/RConn1 -- Chassis/RConn2
  Powertrain/LConn1 -- A1 to World/LConn1 -- Chassis/LConn2
  Powertrain/RConn2 -- Chassis/RConn4 -- A2 to World/LConn1
  Chassis/RConn3 -- Powertrain/RConn1

== system sm_car_/Vehicle/Vehicle Constraint ==
  No Constraint : Subsystem  VariantControl=NoConstraint
  No Yaw : Subsystem  VariantControl=NoYaw
  F : PMIOPort  Side=Right
  B : PMIOPort  Port=2  Side=Left

== system sm_car_/Visualization/Dashboard ==
  VehBus : Inport
  DrvBus : Inport  Port=2
  Accelerator Pedal : LinearGaugeBlock  LabelPosition=Hide  ScaleMax=1  FontColor=[0.0, 0.0, 0.0]
  Brake Pedal : LinearGaugeBlock  ScaleMax=1  FontColor=[0.0, 0.0, 0.0]
  Bus Selector : BusSelector  OutputSignals=Chassis.Body.CG.vx
  Bus Selector2 : BusSelector  OutputSignals=aSteerWheel,rAccelPedal,rBrakePedal
  Gain : Gain  Gain=180/pi
  Gain1 : Gain  Gain=3.6
  Speed (kph) : CustomWebBlock  LabelPosition=Hide  ShowInitialText=on  Configuration="{\"components\":[{\"name\":\"CircularScaleComponent\",\"settings\":{\"bounds\":{\"max\":150,\"min\":0,\"tickInterval\":\"auto\"},\"direction\":\"cw\",\"flipLimits\":0,\"innerRadius\":0.46396628518311167,\"internalTickHeightScaleFactor\":1,\"labelColor\":[250,245,200],\"labelFont\":{\"font\":\"Arial\",\"fontSize\":12},\"labelRadius\":0.36,\"labelTransparency\":1,\"minorTickHeightScaleFactor\":0.2,\"needleImage\":{\"size\":[1890,567],\"src\":\"data:image\\/svg+xml;base64,PD94bWwgdmVyc2lvbj0iMS4wIiBlbmNvZGluZz0iVVRGLTgiIHN0YW5kYWxvbmU9Im5vIj8+CjxzdmcKICAgeG1sbnM6ZGM9Imh0dHA6Ly9wdXJsLm9yZy9kYy9lbGVtZW50cy8xLjEvIgogICB4bWxuczpjYz0iaHR0cDovL2NyZWF0aXZlY29tbW9ucy5vcmcvbnMjIgogICB4bWxuczpyZGY9Imh0dHA6Ly93d3cudzMub3JnLzE5OTkvMDIvMjItcmRmLXN5bnRheC1ucyMiCiAgIHhtbG5zOnN2Zz0iaHR0cDovL3d3dy53My5vcmcvMjAwMC9zdmciCiAgIHhtbG5zPSJodHRwOi8vd3d3LnczLm9yZy8yMDAwL3N2ZyIKICAgeG1sbnM6 ...(+4096 chars)\"},\"needleOffset\":[0.14,0],\"needleOrientation\":-45,\"needleRotation\":180,\"needleSize\":{\"height\":0.13,\"width\":0.41},\"outerRadius\":0.6228849068763098,\"position\":[0,0,1,1],\"referencePoint\":\"auto\",\"scaleAngle\":299.999999999988,\"scaleAngleOffset\":119.46147497096791,\"scaleColors\":[],\"scaleColorsSize\":0.2,\"scaleDirection\":\"CW\",\"scalePosition\":[0,0,1,1],\"showLabels\":1,\"showMinorTicks\":1,\"showSpanLine\":1,\"showTicks\":1,\"tickColor\":[250,245,200],\"tickTransparency\":1,\"valueBarColor\":[23,89,176],\"valueBarPosition\":[0,0,1,1],\"valueBarSize\":0.2,\"valueBarTransparency\":1}},{\"name\":\"BackgroundImageComponent\",\"settings\":{\"image\":{\"size\":[500,500],\"src\":\"data:image\\/svg+xml;base64,PD94bWwgdmVyc2lvbj0iMS4wIiBlbmNvZGluZz0iVVRGLTgiIHN0YW5kYWxvbmU9Im5vIj8+CjwhLS0gR2VuZXJhdG9yOiBBZG9iZSBJbGx1c3RyYXRvciAxOS4yLjEsIFNWRyBFeHBvcnQgUGx1Zy1JbiAuIFNWRyBWZXJzaW9uOiA2LjAwIEJ1aWxkIDApICAtLT4KCjxzdmcKICAgeG1sbnM6ZGM9Imh0dHA6Ly9wdXJsLm9yZy9kYy9lbGVtZW50cy8xLjEvIgogICB4bWxuczpjYz0iaHR0cDovL2NyZWF0aXZlY29tbW9ucy5vcmcvbnMjIgogICB4bWxuczpyZGY9Imh0dHA6Ly93d3cudzMub3JnLzE5OTkvMDIvMjItcmRmLXN5bnRh ...(+9660 chars)\",\"srcOrientation\":\"horizontal\"},\"position\":[0,0,1,1],\"scaleMode\":\"0\"}},{\"name\":\"ForegroundImageComponent\",\"settings\":{\"image\":{\"size\":[0,0],\"src\":\"default\",\"srcOrientation\":[]},\"isForeground\":1,\"position\":[0,0,1,1],\"scaleMode\":\"0\"}}],\"derived\":{\"blockParameters\":{\"ForegroundColor\":[0.9803921568627451,0.9607843137254902,0.7843137254901961],\"Limits\":{\"Max\":150,\"Min\":0,\"Ticks\":\"auto\"},\"ScaleColors\":[],\"ScaleDirection\":\"Clockwise\",\"ScaleMax\":150,\"ScaleMin\":0,\"TickInterval\":\"auto\",\"fixedAspectRatio\":\"on\"}},\"settings\":{\"BindingType\":\"signal\",\"backgroundOffset\":0.14,\"backgroundOpacity\":1,\"fixedAspectRatio\":\"on\",\"orientation\":\"horizontal\",\"showBackgroundColor\":0,\"version\":\"R2024b\"},\"type\":\"CircularGauge\"}"
  Steering Wheel Angle : SemiCircularGaugeBlock  LabelPosition=Hide  ScaleMin=-80  ScaleMax=80  TickInterval=20  FontColor=[0.0, 0.0, 0.0]
  Terminator{,1..3} (4 alike) : Terminator
  wires:
  VehBus/1 -> Bus Selector/1
  DrvBus/1 -> Bus Selector2/1
  Bus Selector/1 -> Gain1/1  "<vx>"
  Gain/1 -> Terminator1/1  "aSteerWheel deg"
  Bus Selector2/3 -> Terminator3/1  "<rBrakePedal>"
  Bus Selector2/1 -> Gain/1  "<aSteerWheel>"
  Bus Selector2/2 -> Terminator2/1  "<rAccelPedal>"
  Gain1/1 -> Terminator/1  "Speed (kph)"
